simulink library "Contact_Forces_Lib"  (R2025a)
settings: Solver=ode45  StartTime=0.0  StopTime=10.0  RelTol=1e-3  EnableMultiTasking=on
undefined symbols (not defined in the file or in its folder): b_contact, custom_param_1, custom_param_2, Extr_Data_Ring, k_contact, l_cone, length_cylinder, length_tube, mu_kinetic, mu_static, pen_exponent, pen_full_damp_F, rad_s_cone, radius_cylinder, radius_tube, v_thr, X, Y, Z
libraries: nesl_utility x197, sm_lib x115, $bdroot x72, simulink x20, fl_lib x4
(part 6 of 12)

== system Contact_Forces_Lib/2D/Circle to Finite Line Force Enabled/Demux ==
  F : Inport
  Bus Creator : BusCreator  Inputs=2
  Bus Creator1 : BusCreator  Inputs=3
  Constant : Constant  Value=0
  Demux : Demux  Outputs=[3 3]
  Demux1 : Demux  Outputs=3
  Demux2 : Demux  Outputs=3
  Gain : Gain  Gain=-1
  Gain1 : Gain
  Simulink-PS Converter{,1..7} (8 alike) : nesl_utility/Simulink-PS Converter  PhysicalDomain=network_engine_domain  SubClassName=ps_input  LeftPortType=input  RightPortType=output  PseudoPeriodic=off  Frequencies=[]  NoiseDistribution=none  NoiseParameters=[]  Unit=1  AffineConversion=off  FilteringAndDerivatives=zero  SimscapeFilterOrder=1  InputFilterTimeConstant=0.005  UdotUserProvided=[]
  Fx Cir : PMIOPort  Side=Right
  Fy Cir : PMIOPort  Port=2  Side=Right
  Fz Cir : PMIOPort  Port=3  Side=Right
  Tz Cir : PMIOPort  Port=4  Side=Right
  Fx Lin : PMIOPort  Port=5  Side=Right
  Fy Lin : PMIOPort  Port=6  Side=Right
  Fz Lin : PMIOPort  Port=7  Side=Right
  Tz Lin : PMIOPort  Port=8  Side=Right
  FCir : Outport  VectorParamsAs1DForOutWhenUnconnected=off
  FLin : Outport  Port=2  VectorParamsAs1DForOutWhenUnconnected=off
  wires:
  Bus Creator1/1 -> FLin/1  "FLin"
  Bus Creator/1 -> FCir/1  "FCir"
  Gain1/1 -> Demux1/1
  F/1 -> Demux/1
  Demux/2 -> Gain/1
  Demux/1 -> Gain1/1
  Demux1/1 -> Simulink-PS Converter/1, Bus Creator/1  "Fx"
  Demux1/2 -> Simulink-PS Converter1/1, Bus Creator/2  "Fy"
  Constant/1 -> Simulink-PS Converter2/1, Simulink-PS Converter5/1
  Demux2/2 -> Simulink-PS Converter4/1, Bus Creator1/2  "Fy"
  Demux2/1 -> Simulink-PS Converter3/1, Bus Creator1/1  "Fx"
  Demux2/3 -> Simulink-PS Converter6/1, Bus Creator1/3  "Tz"
  Demux1/3 -> Simulink-PS Converter7/1
  Gain/1 -> Demux2/1
  connections:
  Fz Cir/RConn1 -- Simulink-PS Converter2/RConn1
  Fy Cir/RConn1 -- Simulink-PS Converter1/RConn1
  Fx Cir/RConn1 -- Simulink-PS Converter/RConn1
  Tz Lin/RConn1 -- Simulink-PS Converter6/RConn1
  Fx Lin/RConn1 -- Simulink-PS Converter3/RConn1
  Fy Lin/RConn1 -- Simulink-PS Converter4/RConn1
  Fz Lin/RConn1 -- Simulink-PS Converter5/RConn1
  Tz Cir/RConn1 -- Simulink-PS Converter7/RConn1

== system Contact_Forces_Lib/2D/Circle to Finite Line Force Enabled/Enable Force ==
  y : Inport
  Abs1 : Abs  ZeroCross=off  SaturateOnIntegerOverflow=off
  Activation limit for contact force : Constant  Value=line_length/2
  Sum : Sum  Inputs=+-
  Enable : Outport  VectorParamsAs1DForOutWhenUnconnected=off
  wires:
  Abs1/1 -> Sum/2
  y/1 -> Abs1/1
  Activation limit for contact force/1 -> Sum/1
  Sum/1 -> Enable/1

== system Contact_Forces_Lib/2D/Circle to Finite Line Force Enabled/Forces ==
  M arm : Inport
  X Sep : Inport  Port=2
  Pos Cmp : Inport  Port=3
  Pen : Inport  Port=4
  Vel : Inport  Port=5
  Vel_Cmp : Inport  Port=6
  Unit Vector : Inport  Port=7
  vy : Inport  Port=8
  wz : Inport  Port=9
  Action Port : ActionPort  ActionPortLabel=if { }
  Force Law : $bdroot/Force Law  SystemSampleTime=-1  LabelModeActiveChoice=Linear  VariantActivationTime=update diagram  EmptyChoice=off  PassThrough=off  PassThroughVariantControl=(default)  EmptyChoiceVariantControl=(default)  AllowFlexibleInterface=on  Latency=0  AutoFrameSizeCalculation=off
  Mux : Mux  Inputs=6
  Resolve Forces : Subsystem
  Subsystem : Subsystem
  Fnf : Outport  InitialOutput=[0]  VectorParamsAs1DForOutWhenUnconnected=off
  F : Outport  Port=2  VectorParamsAs1DForOutWhenUnconnected=off
  wires:
  Subsystem/1(Out) -> Fnf/1
  Resolve Forces/8(Ff) -> Subsystem/2(Ff)
  Resolve Forces/7(Fn) -> Subsystem/1(Fn)
  Resolve Forces/4(Fx Lin) -> Mux/4
  Pen/1 -> Force Law/1
  Vel/1 -> Force Law/2
  Resolve Forces/5(Fy Lin) -> Mux/5
  Resolve Forces/6(Tz Lin) -> Mux/6
  Resolve Forces/1(Fx Cir) -> Mux/1
  Resolve Forces/2(Fy Cir) -> Mux/2
  M arm/1 -> Resolve Forces/1(Moment arm)
  Pos Cmp/1 -> Resolve Forces/2(Pos Cmp)
  Mux/1 -> F/1
  Vel_Cmp/1 -> Resolve Forces/6(Vel Cmp)
  Unit Vector/1 -> Resolve Forces/7(Unit Vector)
  wz/1 -> Resolve Forces/9(wz)
  vy/1 -> Resolve Forces/8(vy)
  Resolve Forces/3(Tz Cir) -> Mux/3
  Force Law/1 -> Resolve Forces/4(Spr Force Mag)
  Force Law/2 -> Resolve Forces/5(Damp Force Mag)
  X Sep/1 -> Resolve Forces/3(X Sep)

== system Contact_Forces_Lib/2D/Circle to Finite Line Force Enabled/No Force ==
  Action Port : ActionPort  ActionPortLabel=else { }
  Zeros : Constant  Value=[0 0 0 0 0 0]  SampleTime=0
  Zeros1 : Constant  Value=[0 0]  SampleTime=0
  Fnf : Outport  InitialOutput=[0]  VectorParamsAs1DForOutWhenUnconnected=off
  F : Outport  Port=2  InitialOutput=[0 0 0 0 0 0]  VectorParamsAs1DForOutWhenUnconnected=off
  wires:
  Zeros1/1 -> Fnf/1
  Zeros/1 -> F/1

== system Contact_Forces_Lib/2D/Circle to Finite Line Force Enabled/Sensing ==
  In : Inport
  Bus Selector : BusSelector  OutputSignals=vy
  PS-Simulink Converter{,1..5} (6 alike) : nesl_utility/PS-Simulink Converter  PhysicalDomain=network_engine_domain  SubClassName=ps_output  LeftPortType=input  RightPortType=output  PseudoPeriodic=off  Frequencies=[]  VectorFormat=1-D array  Unit=1  AffineConversion=off
  Product : Product
  Selector : Selector  NumberOfDimensions=2  InputPortWidth=3  IndexOptions=Index vector (dialog),Index vector (dialog)  Indices=[1],[1,2]  OutputSizes=1,1
  Sign : Signum  ZeroCross=off
  Sum : Sum  Inputs=|+-
  Transform Sensor : sm_lib/Frames and Transforms/Transform Sensor  MeasurementFrame=Base  RotationSequence=XYX  SenseAngle=off  SenseAxis=off  SenseQ=off  SenseR=on  SenseRotationSequence=off  SenseOmegaX=off  SenseOmegaY=off  SenseOmegaZ=on  SenseOmega=off  SenseQDot=off  SenseRDot=off  SenseRotationSequenceDot=off  SenseAlphaX=off  SenseAlphaY=off  SenseAlphaZ=off  SenseAlpha=off  SenseQDDot=off  SenseRDDot=off  SenseX=on  SenseY=on  SenseZ=off  SenseXYZ=off  SenseRad=off  SenseAzim=off  SenseDist=off  SenseInc=off  SenseXDot=on  SenseYDot=on  SenseZDot=off  SenseXYZDot=off  SenseRadDot=off  SenseAzimDot=off  SenseDistDot=off  SenseIncDot=off  SenseXDDot=off  SenseYDDot=off  SenseZDDot=off  SenseXYZDDot=off  SenseRadDDot=off  SenseAzimDDot=off  SenseDistDDot=off  SenseIncDDot=off
  F : PMIOPort  Side=Left
  B : PMIOPort  Port=2  Side=Left
  y : Outport  VectorParamsAs1DForOutWhenUnconnected=off
  x : Outport  Port=2  VectorParamsAs1DForOutWhenUnconnected=off
  vx : Outport  Port=3  VectorParamsAs1DForOutWhenUnconnected=off
  q : Outport  Port=4  VectorParamsAs1DForOutWhenUnconnected=off
  vy : Outport  Port=5  VectorParamsAs1DForOutWhenUnconnected=off
  wz : Outport  Port=6  VectorParamsAs1DForOutWhenUnconnected=off
  wires:
  PS-Simulink Converter1/1 -> y/1
  PS-Simulink Converter2/1 -> vx/1
  PS-Simulink Converter3/1 -> Sum/1
  PS-Simulink Converter4/1 -> wz/1
  PS-Simulink Converter5/1 -> Selector/1
  Selector/1 -> q/1
  Product/1 -> Sum/2
  Sign/1 -> Product/1
  Bus Selector/1 -> Product/2  "<vy>"
  In/1 -> Bus Selector/1
  PS-Simulink Converter/1 -> x/1, Sign/1
  Sum/1 -> vy/1
  connections:
  Transform Sensor/RConn1 -- F/RConn1
  Transform Sensor/LConn1 -- B/RConn1
  PS-Simulink Converter4/LConn1 -- Transform Sensor/RConn3
  PS-Simulink Converter/LConn1 -- Transform Sensor/RConn4
  PS-Simulink Converter1/LConn1 -- Transform Sensor/RConn5
  PS-Simulink Converter2/LConn1 -- Transform Sensor/RConn6
  PS-Simulink Converter3/LConn1 -- Transform Sensor/RConn7
  PS-Simulink Converter5/LConn1 -- Transform Sensor/RConn2

== system Contact_Forces_Lib/2D/Circle to Hole Force/Calculate Penetration ==
  Pos : Inport
  Vel : Inport  Port=2
  Constant : Constant  Value=max_frame_sep
  Dead Zone Outside : DeadZone  LowerValue=-inf  UpperValue=0
  Gain2 : Gain  Gain=-1
  Sum1 : Sum  Inputs=|-+
  Pen : Outport  VectorParamsAs1DForOutWhenUnconnected=off
  Pen Vel : Outport  Port=2  VectorParamsAs1DForOutWhenUnconnected=off
  wires:
  Pos/1 -> Sum1/1
  Sum1/1 -> Dead Zone Outside/1
  Constant/1 -> Sum1/2
  Dead Zone Outside/1 -> Pen/1
  Gain2/1 -> Pen Vel/1
  Vel/1 -> Gain2/1

== system Contact_Forces_Lib/2D/Circle to Hole Force/Sensing ==
  PS-Simulink Converter1 : nesl_utility/PS-Simulink Converter  PhysicalDomain=network_engine_domain  SubClassName=ps_output  LeftPortType=input  RightPortType=output  PseudoPeriodic=off  Frequencies=[]  VectorFormat=1-D array  Unit=deg  AffineConversion=off
  PS-Simulink Converter4 : nesl_utility/PS-Simulink Converter  PhysicalDomain=network_engine_domain  SubClassName=ps_output  LeftPortType=input  RightPortType=output  PseudoPeriodic=off  Frequencies=[]  VectorFormat=1-D array  Unit=1  AffineConversion=off
  PS-Simulink Converter5 : nesl_utility/PS-Simulink Converter  PhysicalDomain=network_engine_domain  SubClassName=ps_output  LeftPortType=input  RightPortType=output  PseudoPeriodic=off  Frequencies=[]  VectorFormat=1-D array  Unit=1  AffineConversion=off
  PS-Simulink Converter6 : nesl_utility/PS-Simulink Converter  PhysicalDomain=network_engine_domain  SubClassName=ps_output  LeftPortType=input  RightPortType=output  PseudoPeriodic=off  Frequencies=[]  VectorFormat=1-D array  Unit=1  AffineConversion=off
  Selector : Selector  NumberOfDimensions=2  InputPortWidth=3  IndexOptions=Index vector (dialog),Index vector (dialog)  Indices=[1],[1,2]  OutputSizes=1,1
  Transform Sensor : sm_lib/Frames and Transforms/Transform Sensor  MeasurementFrame=NonRotatingBase  RotationSequence=XYX  SenseAngle=off  SenseAxis=off  SenseQ=off  SenseR=off  SenseRotationSequence=off  SenseOmegaX=off  SenseOmegaY=off  SenseOmegaZ=off  SenseOmega=off  SenseQDot=off  SenseRDot=off  SenseRotationSequenceDot=off  SenseAlphaX=off  SenseAlphaY=off  SenseAlphaZ=off  SenseAlpha=off  SenseQDDot=off  SenseRDDot=off  SenseX=off  SenseY=off  SenseZ=off  SenseXYZ=off  SenseRad=on  SenseAzim=on  SenseDist=off  SenseInc=off  SenseXDot=off  SenseYDot=off  SenseZDot=off  SenseXYZDot=off  SenseRadDot=on  SenseAzimDot=off  SenseDistDot=off  SenseIncDot=off  SenseXDDot=off  SenseYDDot=off  SenseZDDot=off  SenseXYZDDot=off  SenseRadDDot=off  SenseAzimDDot=off  SenseDistDDot=off  SenseIncDDot=off
  Transform Sensor1 : sm_lib/Frames and Transforms/Transform Sensor  MeasurementFrame=World  RotationSequence=XYX  SenseAngle=off  SenseAxis=off  SenseQ=off  SenseR=on  SenseRotationSequence=off  SenseOmegaX=off  SenseOmegaY=off  SenseOmegaZ=off  SenseOmega=off  SenseQDot=off  SenseRDot=off  SenseRotationSequenceDot=off  SenseAlphaX=off  SenseAlphaY=off  SenseAlphaZ=off  SenseAlpha=off  SenseQDDot=off  SenseRDDot=off  SenseX=off  SenseY=off  SenseZ=off  SenseXYZ=off  SenseRad=off  SenseAzim=off  SenseDist=off  SenseInc=off  SenseXDot=off  SenseYDot=off  SenseZDot=off  SenseXYZDot=off  SenseRadDot=off  SenseAzimDot=off  SenseDistDot=off  SenseIncDot=off  SenseXDDot=off  SenseYDDot=off  SenseZDDot=off  SenseXYZDDot=off  SenseRadDDot=off  SenseAzimDDot=off  SenseDistDDot=off  SenseIncDDot=off
  F : PMIOPort  Side=Left
  B : PMIOPort  Port=2  Side=Left
  rad : Outport  VectorParamsAs1DForOutWhenUnconnected=off
  vrad : Outport  Port=2  VectorParamsAs1DForOutWhenUnconnected=off
  q : Outport  Port=3  VectorParamsAs1DForOutWhenUnconnected=off
  azm : Outport  Port=4  VectorParamsAs1DForOutWhenUnconnected=off
  wires:
  PS-Simulink Converter1/1 -> azm/1
  PS-Simulink Converter5/1 -> rad/1
  PS-Simulink Converter4/1 -> vrad/1
  Selector/1 -> q/1
  PS-Simulink Converter6/1 -> Selector/1
  connections:
  PS-Simulink Converter4/LConn1 -- Transform Sensor/RConn4
  PS-Simulink Converter5/LConn1 -- Transform Sensor/RConn2
  PS-Simulink Converter1/LConn1 -- Transform Sensor/RConn3
  PS-Simulink Converter6/LConn1 -- Transform Sensor1/RConn2
  Transform Sensor1/LConn1 -- B/RConn1 -- Transform Sensor/LConn1
  Transform Sensor1/RConn1 -- Transform Sensor/RConn1 -- F/RConn1

== system Contact_Forces_Lib/2D/Circle to Ring Force/Check Active ==
  Force : Inport
  Active : Inport  Port=2
  PosVel : Inport  Port=3
  Bus Creator : BusCreator  Inputs=7
  Bus Selector : BusSelector  OutputSignals=Normal Force,Friction Force,Penetration,Penetration Vel,Spr Force,Damp Force
  Data Type Conversion : DataTypeConversion  OutDataTypeStr=double  SaturateOnIntegerOverflow=off  RndMeth=Floor
  Demux : Demux  Outputs=6
  Mux : Mux  Inputs=6
  Product : Product
  Out : Outport  VectorParamsAs1DForOutWhenUnconnected=off
  wires:
  Demux/1 -> Bus Creator/1  "Normal Force"
  Demux/2 -> Bus Creator/2  "Friction Force"
  Demux/3 -> Bus Creator/3  "Penetration"
  Demux/6 -> Bus Creator/6  "Damp Force"
  Demux/5 -> Bus Creator/5  "Spr Force"
  Demux/4 -> Bus Creator/4  "Penetration Vel"
  Product/1 -> Demux/1
  Data Type Conversion/1 -> Product/1
  Active/1 -> Data Type Conversion/1
  Mux/1 -> Product/2
  Bus Selector/6 -> Mux/6  "<Damp Force>"
  Bus Creator/1 -> Out/1
  Force/1 -> Bus Selector/1
  Bus Selector/5 -> Mux/5  "<Spr Force>"
  Bus Selector/3 -> Mux/3  "<Penetration>"
  Bus Selector/4 -> Mux/4  "<Penetration Vel>"
  PosVel/1 -> Bus Creator/7
  Bus Selector/2 -> Mux/2  "<Friction Force>"
  Bus Selector/1 -> Mux/1  "<Normal Force>"

== system Contact_Forces_Lib/2D/Circle to Ring Force/Check Active Range ==
  azm : Inport
  " Upper Bound" : simulink/Logic and Bit Operations/Compare To Constant  relop=<=  const=active_angle(2)  OutDataTypeStr=boolean  ZeroCross=off
  Logical Operator : Logic  AllPortsSameDT=off  OutDataTypeStr=boolean
  Lower Bound : simulink/Logic and Bit Operations/Compare To Constant  relop=>=  const=active_angle(1)  OutDataTypeStr=boolean  ZeroCross=off
  En : Outport  VectorParamsAs1DForOutWhenUnconnected=off
  wires:
  azm/1 -> " Upper Bound"/1, Lower Bound/1
  " Upper Bound"/1 -> Logical Operator/1
  Logical Operator/1 -> En/1
  Lower Bound/1 -> Logical Operator/2

== system Contact_Forces_Lib/2D/Circle to Ring Force/Forces ==
  rad : Inport
  vrad : Inport  Port=2
  azm : Inport  Port=3
  vazm : Inport  Port=4
  wzf : Inport  Port=5
  R : Inport  Port=6
  Action Port : ActionPort
  Bus Creator : BusCreator  Inputs=6
  Calculate Penetration : Subsystem
  Ff : Subsystem
  Fn : Subsystem
  Force Law : $bdroot/Force Law  SystemSampleTime=-1  LabelModeActiveChoice=Linear  VariantActivationTime=update diagram  EmptyChoice=off  PassThrough=off  PassThroughVariantControl=(default)  EmptyChoiceVariantControl=(default)  AllowFlexibleInterface=on  Latency=0  AutoFrameSizeCalculation=off
  Gain1 : Gain  Gain=-1
  Mux : Mux  Inputs=6
  Product : Product
  Sum : Subsystem
  Sum1 : Sum  Inputs=+-
  Frc : Outport  VectorParamsAs1DForOutWhenUnconnected=off
  Out : Outport  Port=2  InitialOutput=[0]  VectorParamsAs1DForOutWhenUnconnected=off
  wires:
  Bus Creator/1 -> Out/1
  Force Law/1 -> Bus Creator/4, Sum1/1  "Spr Force"
  Calculate Penetration/3(Pen Vel) -> Bus Creator/1, Force Law/2  "Penetration Vel"
  vrad/1 -> Calculate Penetration/2(vrad)
  rad/1 -> Ff/7(rad), Calculate Penetration/1(rad)
  Product/1 -> Bus Creator/5, Gain1/1  "Normal Force"
  Calculate Penetration/2(Pen) -> Bus Creator/2, Ff/6(Pen), Force Law/1  "Penetration"
  Calculate Penetration/1(sign) -> Product/1
  Force Law/2 -> Bus Creator/3, Sum1/2  "Damp Force"
  Sum1/1 -> Product/2
  Gain1/1 -> Ff/5(Fn), Fn/1(Fn)
  R/1 -> Ff/1(R), Fn/2(R)
  azm/1 -> Fn/3(azm), Ff/2(azm)
  vazm/1 -> Ff/3(vazm)
  wzf/1 -> Ff/4(wzf)
  Fn/1(FxCirF) -> Sum/1(FnxCirF)
  Fn/2(FyCirF) -> Sum/2(FnyCirF)
  Fn/3(FxCirB) -> Sum/3(FnxCirB)
  Fn/4(FyCirB) -> Sum/4(FnyCirB)
  Ff/4(FyCirB) -> Sum/8(FfyCirB)
  Ff/6(TzCirB) -> Sum/10(TzCirB)
  Ff/3(FxCirB) -> Sum/7(FfxCirB)
  Ff/5(TzCirF) -> Sum/9(TzCirF)
  Ff/1(FxCirF) -> Sum/5(FfxCirF)
  Ff/2(FyCirF) -> Sum/6(FfyCirF)
  Sum/2(FyF) -> Mux/2
  Sum/3(TzF) -> Mux/3
  Sum/1(FxF) -> Mux/1
  Sum/5(FyB) -> Mux/5
  Sum/4(FxB) -> Mux/4
  Sum/6(TzB) -> Mux/6
  Mux/1 -> Frc/1
  Ff/7(Ff) -> Bus Creator/6  "Friction Force"

== system Contact_Forces_Lib/2D/Circle to Ring Force/No Force ==
  Action Port : ActionPort
  Zeros : Constant  Value=[0 0 0 0 0 0]  SampleTime=0
  F : Outport  InitialOutput=[0]  VectorParamsAs1DForOutWhenUnconnected=off
  wires:
  Zeros/1 -> F/1

== system Contact_Forces_Lib/2D/Circle to Ring Force/Sensing ==
  PS-Simulink Converter1 : nesl_utility/PS-Simulink Converter  PhysicalDomain=network_engine_domain  SubClassName=ps_output  LeftPortType=input  RightPortType=output  PseudoPeriodic=off  Frequencies=[]  VectorFormat=1-D array  Unit=deg  AffineConversion=off
  PS-Simulink Converter{2..6} (5 alike) : nesl_utility/PS-Simulink Converter  PhysicalDomain=network_engine_domain  SubClassName=ps_output  LeftPortType=input  RightPortType=output  PseudoPeriodic=off  Frequencies=[]  VectorFormat=1-D array  Unit=1  AffineConversion=off
  Selector : Selector  NumberOfDimensions=2  InputPortWidth=3  IndexOptions=Index vector (dialog),Index vector (dialog)  Indices=[1,2],[1,2]  OutputSizes=1,1
  Transform Sensor Base : sm_lib/Frames and Transforms/Transform Sensor  MeasurementFrame=Base  RotationSequence=XYX  SenseAngle=off  SenseAxis=off  SenseQ=off  SenseR=on  SenseRotationSequence=off  SenseOmegaX=off  SenseOmegaY=off  SenseOmegaZ=on  SenseOmega=off  SenseQDot=off  SenseRDot=off  SenseRotationSequenceDot=off  SenseAlphaX=off  SenseAlphaY=off  SenseAlphaZ=off  SenseAlpha=off  SenseQDDot=off  SenseRDDot=off  SenseX=off  SenseY=off  SenseZ=off  SenseXYZ=off  SenseRad=on  SenseAzim=on  SenseDist=off  SenseInc=off  SenseXDot=off  SenseYDot=off  SenseZDot=off  SenseXYZDot=off  SenseRadDot=on  SenseAzimDot=on  SenseDistDot=off  SenseIncDot=off  SenseXDDot=off  SenseYDDot=off  SenseZDDot=off  SenseXYZDDot=off  SenseRadDDot=off  SenseAzimDDot=off  SenseDistDDot=off  SenseIncDDot=off
  F : PMIOPort  Side=Left
  B : PMIOPort  Port=2  Side=Left
  rad : Outport  VectorParamsAs1DForOutWhenUnconnected=off
  vrad : Outport  Port=2  VectorParamsAs1DForOutWhenUnconnected=off
  azm : Outport  Port=3  VectorParamsAs1DForOutWhenUnconnected=off
  vazm : Outport  Port=4  VectorParamsAs1DForOutWhenUnconnected=off
  wzf : Outport  Port=5  VectorParamsAs1DForOutWhenUnconnected=off
  R : Outport  Port=6  VectorParamsAs1DForOutWhenUnconnected=off
  wires:
  PS-Simulink Converter3/1 -> wzf/1
  PS-Simulink Converter2/1 -> vazm/1
  PS-Simulink Converter6/1 -> Selector/1
  Selector/1 -> R/1
  PS-Simulink Converter4/1 -> vrad/1
  PS-Simulink Converter5/1 -> rad/1
  PS-Simulink Converter1/1 -> azm/1
  connections:
  PS-Simulink Converter2/LConn1 -- Transform Sensor Base/RConn7
  F/RConn1 -- Transform Sensor Base/RConn1
  Transform Sensor Base/LConn1 -- B/RConn1
  PS-Simulink Converter6/LConn1 -- Transform Sensor Base/RConn2
  PS-Simulink Converter1/LConn1 -- Transform Sensor Base/RConn5
  PS-Simulink Converter5/LConn1 -- Transform Sensor Base/RConn4
  PS-Simulink Converter4/LConn1 -- Transform Sensor Base/RConn6
  PS-Simulink Converter3/LConn1 -- Transform Sensor Base/RConn3

== system Contact_Forces_Lib/2D/Circle to Ring Force/Subsystem ==
  Frc : Inport
  Demux : Demux  Outputs=6
  Simulink-PS Converter{,1..5} (6 alike) : nesl_utility/Simulink-PS Converter  PhysicalDomain=network_engine_domain  SubClassName=ps_input  LeftPortType=input  RightPortType=output  PseudoPeriodic=off  Frequencies=[]  NoiseDistribution=none  NoiseParameters=[]  Unit=1  AffineConversion=off  FilteringAndDerivatives=zero  SimscapeFilterOrder=1  InputFilterTimeConstant=0.005  UdotUserProvided=1
  FxF : PMIOPort  Side=Right
  FyF : PMIOPort  Port=2  Side=Right
  TzF : PMIOPort  Port=3  Side=Right
  FxB : PMIOPort  Port=4  Side=Right
  FyB : PMIOPort  Port=5  Side=Right
  TzB : PMIOPort  Port=6  Side=Right
  wires:
  Frc/1 -> Demux/1
  Demux/6 -> Simulink-PS Converter5/1
  Demux/5 -> Simulink-PS Converter4/1
  Demux/4 -> Simulink-PS Converter3/1
  Demux/3 -> Simulink-PS Converter2/1
  Demux/1 -> Simulink-PS Converter/1
  Demux/2 -> Simulink-PS Converter1/1
  connections:
  Simulink-PS Converter2/RConn1 -- TzF/RConn1
  Simulink-PS Converter4/RConn1 -- FyB/RConn1
  Simulink-PS Converter3/RConn1 -- FxB/RConn1
  Simulink-PS Converter5/RConn1 -- TzB/RConn1
  Simulink-PS Converter/RConn1 -- FxF/RConn1
  Simulink-PS Converter1/RConn1 -- FyF/RConn1

== system Contact_Forces_Lib/2D/Composite Forces/Box to Belt Force ==
  Spd : Inport
  Add2 : Sum
  Belt Ends : Subsystem
      mask Display:
      | image(imread('Box_to_Belt_Ends_IMAGE.jpg'));
      | port_label('LConn',1,'Bel');
      | port_label('RConn',1,'Box');
      | port_label('input',1,'In');
      | port_label('output',1,'Fn');
  Belt Faces : Subsystem
      mask Display:
      | image(imread('Box_to_Belt_Faces_IMAGE.jpg'));
      | port_label('LConn',1,'Bel');
      | port_label('RConn',1,'Box');
      | port_label('input',1,'In');
      | port_label('output',1,'Fn');
  Bus Creator : BusCreator  Inputs=2
  Enable : Constant
  Box : PMIOPort  Side=Right
  Bel : PMIOPort  Port=2  Side=Left
  Fn : Outport  VectorParamsAs1DForOutWhenUnconnected=off
  wires:
  Belt Faces/1(Fn) -> Add2/1
  Belt Ends/1(Fn) -> Add2/2
  Add2/1 -> Fn/1
  Enable/1 -> Bus Creator/1  "Enable"
  Spd/1 -> Bus Creator/2  "vy"
  Bus Creator/1 -> Belt Ends/1(In), Belt Faces/1(In1)
  connections:
  Belt Faces/LConn1 -- Bel/RConn1 -- Belt Ends/LConn1
  Belt Faces/RConn1 -- Box/RConn1 -- Belt Ends/RConn1

== system Contact_Forces_Lib/2D/Composite Forces/Box to Box Force ==
  Abs : Abs  ZeroCross=off  SaturateOnIntegerOverflow=off
  Abs1 : Abs  ZeroCross=off  SaturateOnIntegerOverflow=off
  Add : Sum
  BoxB Corners : Subsystem  mask(Contact Forces, Base Box Corners){}
      mask help:
      | This subsystem models planar contact forces the corners of the Follower box and the faces of the Base Box.
      |
      | Click the Help button for a diagram of the contact forces and the parameters.
      mask Help: web(which('Box_to_Box_Contact_Forces_BoxB_Corners.html'));
      mask Display:
      | image(imread('BoxB_Corners_IMAGE.jpg'));
      | port_label('LConn',1,'BoxB');
      | port_label('RConn',1,'BoxF');
  BoxF Corners : Subsystem  mask(Contact Forces, Follower Box Corners){}
      mask help:
      | This subsystem models planar contact forces the corners of the Follower box and the faces of the Base Box.
      |
      | Click the Help button for a diagram of the contact forces and the parameters.
      mask Help: web(which('Box_to_Box_Contact_Forces_BoxF_Corners.html'));
      mask Display:
      | image(imread('BoxF_Corners_IMAGE.jpg'));
      | port_label('LConn',1,'BoxB');
      | port_label('RConn',1,'BoxF');
  Goto Tag Visibility : GotoTagVisibility  GotoTag=FrcFC
  Goto Tag Visibility1 : GotoTagVisibility  GotoTag=FrcBC
  Sum of Elements : Sum  Inputs=+
  Sum of Elements1 : Sum  Inputs=+
  BoxF : PMIOPort  Side=Left
  BoxB : PMIOPort  Port=2  Side=Right
  Out : Outport  VectorParamsAs1DForOutWhenUnconnected=off
  wires:
  Sum of Elements1/1 -> Add/2
  Add/1 -> Out/1
  Abs1/1 -> Sum of Elements1/1
  [FrcBC] -> Abs1/1
  Abs/1 -> Sum of Elements/1
  Sum of Elements/1 -> Add/1
  [FrcFC] -> Abs/1
  connections:
  BoxB Corners/LConn1 -- BoxF Corners/LConn1 -- BoxB/RConn1
  BoxB Corners/RConn1 -- BoxF Corners/RConn1 -- BoxF/RConn1

== system Contact_Forces_Lib/3D/Composite Forces/Face to Belt Faces Force ==
  In : Inport
  Bus Creator : BusCreator  Inputs=4
  Sphere to Plane Force Enabled nz{1..4} (4 alike) : $bdroot/3D/Sphere to Plane Force Enabled  sphere_rad=FacF_rSph  plane_lenx=PlaB_x  plane_leny=PlaB_y  plane_depth=PlaB_z  force_law=Linear  k_contact=k_contact_pla2pla  b_contact=b_contact_pla2pla  pen_full_damp_F=pen_full_damp_F_pla2pla  pen_exponent=pen_exponent_pla2pla  custom_param_1=1  custom_param_2=1  friction_law=Stick-Slip Continuous  mu_kinetic=mu_kinetic_pla2pla  mu_static=mu_static_pla2pla  v_thr=v_thr_pla2pla  vis_on=off  vis_opc_en=0  vis_len_plaBz=vis_len_plaLz  vis_clr=vis_clr  vis_opc=vis_opc
  Transform Fnz1 : sm_lib/Frames and Transforms/Rigid Transform  RotationMethod=None  FollAlignAxisA=+X  BaseAlignAxisA=+Y  FollAlignAxisB=+Y  BaseAlignAxisB=+Z  RotationStandardAxis=+Z  RotationAngle=0.0  RotationAngleUnits=deg  RotationArbitraryAxis=[0 0 1]  RotationSequenceAxes=FollowerAxes  RotationSequence=XYX  RotationSequenceAngles=[0 0 0]  RotationSequenceAnglesUnits=deg  RotationMatrix=[1 0 0; 0 1 0; 0 0 1]  Quaternion=[1 0 0 0]  TranslationMethod=Cartesian  TranslationCartesianOffset=[FacF_x/2 FacF_y/2 -FacF_z]+[-1 -1 1*sign(FacF_z)]*FacF_rSph  TranslationCartesianOffsetUnits=m  TranslationStandardAxis=-Z  TranslationStandardOffset=0  TranslationStandardOffsetUnits=m  TranslationROffset=0  TranslationROffsetUnits=m  TranslationThetaOffset=0  TranslationThetaOffsetUnits=deg  TranslationZOffset=0  TranslationZOffsetUnits=m
  Transform Fnz2 : sm_lib/Frames and Transforms/Rigid Transform  RotationMethod=None  FollAlignAxisA=+X  BaseAlignAxisA=+Y  FollAlignAxisB=+Y  BaseAlignAxisB=+Z  RotationStandardAxis=+Z  RotationAngle=0.0  RotationAngleUnits=deg  RotationArbitraryAxis=[0 0 1]  RotationSequenceAxes=FollowerAxes  RotationSequence=XYX  RotationSequenceAngles=[0 0 0]  RotationSequenceAnglesUnits=deg  RotationMatrix=[1 0 0; 0 1 0; 0 0 1]  Quaternion=[1 0 0 0]  TranslationMethod=Cartesian  TranslationCartesianOffset=[FacF_x/2 -FacF_y/2 -FacF_z]+[-1 1 1*sign(FacF_z)]*FacF_rSph  TranslationCartesianOffsetUnits=m  TranslationStandardAxis=-Z  TranslationStandardOffset=0  TranslationStandardOffsetUnits=m  TranslationROffset=0  TranslationROffsetUnits=m  TranslationThetaOffset=0  TranslationThetaOffsetUnits=deg  TranslationZOffset=0  TranslationZOffsetUnits=m
  Transform Fnz3 : sm_lib/Frames and Transforms/Rigid Transform  RotationMethod=None  FollAlignAxisA=+X  BaseAlignAxisA=+Y  FollAlignAxisB=+Y  BaseAlignAxisB=+Z  RotationStandardAxis=+Z  RotationAngle=0.0  RotationAngleUnits=deg  RotationArbitraryAxis=[0 0 1]  RotationSequenceAxes=FollowerAxes  RotationSequence=XYX  RotationSequenceAngles=[0 0 0]  RotationSequenceAnglesUnits=deg  RotationMatrix=[1 0 0; 0 1 0; 0 0 1]  Quaternion=[1 0 0 0]  TranslationMethod=Cartesian  TranslationCartesianOffset=[-FacF_x/2 -FacF_y/2 -FacF_z]+[1 1 1*sign(FacF_z)]*FacF_rSph  TranslationCartesianOffsetUnits=m  TranslationStandardAxis=-Z  TranslationStandardOffset=0  TranslationStandardOffsetUnits=m  TranslationROffset=0  TranslationROffsetUnits=m  TranslationThetaOffset=0  TranslationThetaOffsetUnits=deg  TranslationZOffset=0  TranslationZOffsetUnits=m
  Transform Fnz4 : sm_lib/Frames and Transforms/Rigid Transform  RotationMethod=None  FollAlignAxisA=+X  BaseAlignAxisA=+Y  FollAlignAxisB=+Y  BaseAlignAxisB=+Z  RotationStandardAxis=+Z  RotationAngle=0.0  RotationAngleUnits=deg  RotationArbitraryAxis=[0 0 1]  RotationSequenceAxes=FollowerAxes  RotationSequence=XYX  RotationSequenceAngles=[0 0 0]  RotationSequenceAnglesUnits=deg  RotationMatrix=[1 0 0; 0 1 0; 0 0 1]  Quaternion=[1 0 0 0]  TranslationMethod=Cartesian  TranslationCartesianOffset=[-FacF_x/2 FacF_y/2 -FacF_z]+[1 -1 1*sign(FacF_z)]*FacF_rSph  TranslationCartesianOffsetUnits=m  TranslationStandardAxis=-Z  TranslationStandardOffset=0  TranslationStandardOffsetUnits=m  TranslationROffset=0  TranslationROffsetUnits=m  TranslationThetaOffset=0  TranslationThetaOffsetUnits=deg  TranslationZOffset=0  TranslationZOffsetUnits=m
  PlaB : PMIOPort  Side=Right
  FacF : PMIOPort  Port=2  Side=Left
  Out : Outport  VectorParamsAs1DForOutWhenUnconnected=off
  wires:
  In/1 -> Sphere to Plane Force Enabled nz4/1, Sphere to Plane Force Enabled nz3/1, Sphere to Plane Force Enabled nz2/1, Sphere to Plane Force Enabled nz1/1
  Bus Creator/1 -> Out/1
  Sphere to Plane Force Enabled nz3/1 -> Bus Creator/3  "fz3"
  Sphere to Plane Force Enabled nz1/1 -> Bus Creator/1  "fz1"
  Sphere to Plane Force Enabled nz2/1 -> Bus Creator/2  "fz2"
  Sphere to Plane Force Enabled nz4/1 -> Bus Creator/4  "fz4"
  connections:
  Sphere to Plane Force Enabled nz3/LConn1 -- Transform Fnz3/RConn1
  Sphere to Plane Force Enabled nz2/LConn1 -- Transform Fnz2/RConn1
  Sphere to Plane Force Enabled nz4/LConn1 -- Transform Fnz4/RConn1
  Sphere to Plane Force Enabled nz1/LConn1 -- Transform Fnz1/RConn1
  Sphere to Plane Force Enabled nz4/RConn1 -- Sphere to Plane Force Enabled nz2/RConn1 -- Sphere to Plane Force Enabled nz1/RConn1 -- PlaB/RConn1 -- Sphere to Plane Force Enabled nz3/RConn1
  Transform Fnz1/LConn1 -- Transform Fnz3/LConn1 -- Transform Fnz4/LConn1 -- FacF/RConn1 -- Transform Fnz2/LConn1

== system Contact_Forces_Lib/3D/Composite Forces/Face to Plane Force ==
  Bus Creator : BusCreator  Inputs=4
  Sphere to Plane Force nz{1..4} (4 alike) : $bdroot/3D/Sphere to Plane Force  sphere_rad=FacF_rSph  plane_lenx=PlaB_x  plane_leny=PlaB_y  plane_depth=PlaB_z  force_law=Linear  k_contact=k_contact_pla2pla  b_contact=b_contact_pla2pla  pen_full_damp_F=pen_full_damp_F_pla2pla  pen_exponent=pen_exponent_pla2pla  custom_param_1=1  custom_param_2=1  friction_law=None  mu_kinetic=mu_kinetic_pla2pla  mu_static=mu_static_pla2pla  v_thr=v_thr_pla2pla  vis_on=off  vis_opc_en=0  vis_len_plaBz=vis_len_plaLz  vis_clr=vis_clr  vis_opc=vis_opc
  Transform Fnz1 : sm_lib/Frames and Transforms/Rigid Transform  RotationMethod=None  FollAlignAxisA=+X  BaseAlignAxisA=+Y  FollAlignAxisB=+Y  BaseAlignAxisB=+Z  RotationStandardAxis=+Z  RotationAngle=0.0  RotationAngleUnits=deg  RotationArbitraryAxis=[0 0 1]  RotationSequenceAxes=FollowerAxes  RotationSequence=XYX  RotationSequenceAngles=[0 0 0]  RotationSequenceAnglesUnits=deg  RotationMatrix=[1 0 0; 0 1 0; 0 0 1]  Quaternion=[1 0 0 0]  TranslationMethod=Cartesian  TranslationCartesianOffset=[FacF_x/2 FacF_y/2 -FacF_z]+[-1 -1 1*sign(FacF_z)]*FacF_rSph  TranslationCartesianOffsetUnits=m  TranslationStandardAxis=-Z  TranslationStandardOffset=0  TranslationStandardOffsetUnits=m  TranslationROffset=0  TranslationROffsetUnits=m  TranslationThetaOffset=0  TranslationThetaOffsetUnits=deg  TranslationZOffset=0  TranslationZOffsetUnits=m
  Transform Fnz2 : sm_lib/Frames and Transforms/Rigid Transform  RotationMethod=None  FollAlignAxisA=+X  BaseAlignAxisA=+Y  FollAlignAxisB=+Y  BaseAlignAxisB=+Z  RotationStandardAxis=+Z  RotationAngle=0.0  RotationAngleUnits=deg  RotationArbitraryAxis=[0 0 1]  RotationSequenceAxes=FollowerAxes  RotationSequence=XYX  RotationSequenceAngles=[0 0 0]  RotationSequenceAnglesUnits=deg  RotationMatrix=[1 0 0; 0 1 0; 0 0 1]  Quaternion=[1 0 0 0]  TranslationMethod=Cartesian  TranslationCartesianOffset=[FacF_x/2 -FacF_y/2 -FacF_z]+[-1 1 1*sign(FacF_z)]*FacF_rSph  TranslationCartesianOffsetUnits=m  TranslationStandardAxis=-Z  TranslationStandardOffset=0  TranslationStandardOffsetUnits=m  TranslationROffset=0  TranslationROffsetUnits=m  TranslationThetaOffset=0  TranslationThetaOffsetUnits=deg  TranslationZOffset=0  TranslationZOffsetUnits=m
  Transform Fnz3 : sm_lib/Frames and Transforms/Rigid Transform  RotationMethod=None  FollAlignAxisA=+X  BaseAlignAxisA=+Y  FollAlignAxisB=+Y  BaseAlignAxisB=+Z  RotationStandardAxis=+Z  RotationAngle=0.0  RotationAngleUnits=deg  RotationArbitraryAxis=[0 0 1]  RotationSequenceAxes=FollowerAxes  RotationSequence=XYX  RotationSequenceAngles=[0 0 0]  RotationSequenceAnglesUnits=deg  RotationMatrix=[1 0 0; 0 1 0; 0 0 1]  Quaternion=[1 0 0 0]  TranslationMethod=Cartesian  TranslationCartesianOffset=[-FacF_x/2 -FacF_y/2 -FacF_z]+[1 1 1*sign(FacF_z)]*FacF_rSph  TranslationCartesianOffsetUnits=m  TranslationStandardAxis=-Z  TranslationStandardOffset=0  TranslationStandardOffsetUnits=m  TranslationROffset=0  TranslationROffsetUnits=m  TranslationThetaOffset=0  TranslationThetaOffsetUnits=deg  TranslationZOffset=0  TranslationZOffsetUnits=m
  Transform Fnz4 : sm_lib/Frames and Transforms/Rigid Transform  RotationMethod=None  FollAlignAxisA=+X  BaseAlignAxisA=+Y  FollAlignAxisB=+Y  BaseAlignAxisB=+Z  RotationStandardAxis=+Z  RotationAngle=0.0  RotationAngleUnits=deg  RotationArbitraryAxis=[0 0 1]  RotationSequenceAxes=FollowerAxes  RotationSequence=XYX  RotationSequenceAngles=[0 0 0]  RotationSequenceAnglesUnits=deg  RotationMatrix=[1 0 0; 0 1 0; 0 0 1]  Quaternion=[1 0 0 0]  TranslationMethod=Cartesian  TranslationCartesianOffset=[-FacF_x/2 FacF_y/2 -FacF_z]+[1 -1 1*sign(FacF_z)]*FacF_rSph  TranslationCartesianOffsetUnits=m  TranslationStandardAxis=-Z  TranslationStandardOffset=0  TranslationStandardOffsetUnits=m  TranslationROffset=0  TranslationROffsetUnits=m  TranslationThetaOffset=0  TranslationThetaOffsetUnits=deg  TranslationZOffset=0  TranslationZOffsetUnits=m
  PlaB : PMIOPort  Side=Right
  FacF : PMIOPort  Port=2  Side=Left
  Out : Outport  VectorParamsAs1DForOutWhenUnconnected=off
  wires:
  Sphere to Plane Force nz4/1 -> Bus Creator/4  "fz4"
  Sphere to Plane Force nz2/1 -> Bus Creator/2  "fz2"
  Sphere to Plane Force nz1/1 -> Bus Creator/1  "fz1"
  Sphere to Plane Force nz3/1 -> Bus Creator/3  "fz3"
  Bus Creator/1 -> Out/1
  connections:
  FacF/RConn1 -- Transform Fnz1/LConn1 -- Transform Fnz2/LConn1 -- Transform Fnz4/LConn1 -- Transform Fnz3/LConn1
  Sphere to Plane Force nz4/RConn1 -- Sphere to Plane Force nz3/RConn1 -- PlaB/RConn1 -- Sphere to Plane Force nz2/RConn1 -- Sphere to Plane Force nz1/RConn1
  Sphere to Plane Force nz1/LConn1 -- Transform Fnz1/RConn1
  Sphere to Plane Force nz4/LConn1 -- Transform Fnz4/RConn1
  Sphere to Plane Force nz2/LConn1 -- Transform Fnz2/RConn1
  Sphere to Plane Force nz3/LConn1 -- Transform Fnz3/RConn1

== system Contact_Forces_Lib/3D/Composite Forces/Sphere to Belt Force ==
  In : Inport
  Bus Creator : BusCreator  Inputs=3
  Force BeltF to Sph : $bdroot/3D/Sphere to Tube Force Enabled  radius_sphere=sph_rad  radius_tube=belt_h/2*0.8  d_tube=belt_h*0.2  l_tube=belt_w  active_angle=[-90 90]  force_law=Linear  k_contact=k_contact_sph2bel  b_contact=b_contact_sph2bel  pen_full_damp_F=pen_full_damp_F_sph2bel  pen_exponent=pen_exponent_sph2bel  custom_param_1=1  custom_param_2=1  friction_law=Stick-Slip Continuous  mu_kinetic=mu_kinetic_sph2bel  mu_static=mu_static_sph2bel  v_thr=v_thr_sph2bel  vis_on=off  vis_opc_en=0  vis_len_tubBx=vis_depth_sph2bel  vis_clr=vis_clr  vis_opc=vis_opc
  Force BeltM to Sph : $bdroot/3D/Sphere to Plane Force Enabled  sphere_rad=sph_rad  plane_lenx=belt_l  plane_leny=belt_w  plane_depth=belt_h/2  force_law=Linear  k_contact=k_contact_sph2bel  b_contact=b_contact_sph2bel  pen_full_damp_F=pen_full_damp_F_sph2bel  pen_exponent=pen_exponent_sph2bel  custom_param_1=1  custom_param_2=1  friction_law=Stick-Slip Continuous  mu_kinetic=mu_kinetic_sph2bel  mu_static=mu_static_sph2bel  v_thr=v_thr_sph2bel  vis_on=off  vis_opc_en=0  vis_len_plaBz=vis_depth_sph2bel  vis_clr=vis_clr  vis_opc=vis_opc
  Force BeltR to Sph : $bdroot/3D/Sphere to Tube Force Enabled  radius_sphere=sph_rad  radius_tube=belt_h/2*0.8  d_tube=belt_h*0.2  l_tube=belt_w  active_angle=[-90 90]  force_law=Linear  k_contact=k_contact_sph2bel  b_contact=b_contact_sph2bel  pen_full_damp_F=pen_full_damp_F_sph2bel  pen_exponent=pen_exponent_sph2bel  custom_param_1=1  custom_param_2=1  friction_law=Stick-Slip Continuous  mu_kinetic=mu_kinetic_sph2bel  mu_static=mu_static_sph2bel  v_thr=v_thr_sph2bel  vis_on=off  vis_opc_en=0  vis_len_tubBx=vis_depth_sph2bel  vis_clr=vis_clr  vis_opc=vis_opc
  Transform Front : sm_lib/Frames and Transforms/Rigid Transform  RotationMethod=StandardAxis  FollAlignAxisA=+X  BaseAlignAxisA=+Y  FollAlignAxisB=+Y  BaseAlignAxisB=+Z  RotationStandardAxis=+X  RotationAngle=-90  RotationAngleUnits=deg  RotationArbitraryAxis=[0 0 1]  RotationSequenceAxes=FollowerAxes  RotationSequence=XYX  RotationSequenceAngles=[0 0 0]  RotationSequenceAnglesUnits=deg  RotationMatrix=[1 0 0; 0 1 0; 0 0 1]  Quaternion=[1 0 0 0]  TranslationMethod=StandardAxis  TranslationCartesianOffset=[0 0 0]  TranslationCartesianOffsetUnits=m  TranslationStandardAxis=+X  TranslationStandardOffset=belt_l/2  TranslationStandardOffsetUnits=m  TranslationROffset=0  TranslationROffsetUnits=m  TranslationThetaOffset=0  TranslationThetaOffsetUnits=deg  TranslationZOffset=0  TranslationZOffsetUnits=m
  Transform Rear : sm_lib/Frames and Transforms/Rigid Transform  RotationMethod=RotationSequence  FollAlignAxisA=+X  BaseAlignAxisA=+Y  FollAlignAxisB=+Y  BaseAlignAxisB=+Z  RotationStandardAxis=+Y  RotationAngle=180  RotationAngleUnits=deg  RotationArbitraryAxis=[0 0 1]  RotationSequenceAxes=FollowerAxes  RotationSequence=XZX  RotationSequenceAngles=[-90 180 0]  RotationSequenceAnglesUnits=deg  RotationMatrix=[1 0 0; 0 1 0; 0 0 1]  Quaternion=[1 0 0 0]  TranslationMethod=StandardAxis  TranslationCartesianOffset=[0 0 0]  TranslationCartesianOffsetUnits=m  TranslationStandardAxis=+X  TranslationStandardOffset=-belt_l/2  TranslationStandardOffsetUnits=m  TranslationROffset=0  TranslationROffsetUnits=m  TranslationThetaOffset=0  TranslationThetaOffsetUnits=deg  TranslationZOffset=0  TranslationZOffsetUnits=m
  SphF : PMIOPort  Side=Left
  BelB : PMIOPort  Port=2  Side=Right
  Out : Outport  VectorParamsAs1DForOutWhenUnconnected=off
  wires:
  Bus Creator/1 -> Out/1
  Force BeltR to Sph/1 -> Bus Creator/3  "fRea"
  Force BeltM to Sph/1 -> Bus Creator/2  "fMid"
  In/1 -> Force BeltF to Sph/1, Force BeltM to Sph/1, Force BeltR to Sph/1
  Force BeltF to Sph/1 -> Bus Creator/1  "fFro"
  connections:
  Force BeltR to Sph/RConn1 -- Transform Rear/RConn1
  Transform Rear/LConn1 -- Force BeltM to Sph/RConn1 -- Transform Front/LConn1 -- BelB/RConn1
  Transform Front/RConn1 -- Force BeltF to Sph/RConn1
  Force BeltR to Sph/LConn1 -- Force BeltF to Sph/LConn1 -- Force BeltM to Sph/LConn1 -- SphF/RConn1

== system Contact_Forces_Lib/3D/Prototype/Cone in Ring Force ==
  Enable : Subsystem
  External Force and Torque : sm_lib/Forces and Torques/External Force and Torque  EnableForceX=off  EnableForceY=off  EnableForceZ=off  EnableForce=on  ForceResolutionFrame=AttachedFrame  EnableTorqueX=off  EnableTorqueY=off  EnableTorqueZ=off  EnableTorque=on  TorqueResolutionFrame=AttachedFrame
  If : If  IfExpression=u1
  If Action Subsystem : Subsystem  TreatAsAtomicUnit=on
  Merge : Merge
  Merge1 : Merge
  PS-Simulink Converter{1..3,5} (4 alike) : nesl_utility/PS-Simulink Converter  PhysicalDomain=network_engine_domain  SubClassName=ps_output  LeftPortType=input  RightPortType=output  PseudoPeriodic=off  Frequencies=[]  VectorFormat=1-D array  Unit=1  AffineConversion=off
  Point of Contact calc : Subsystem
  Simulink-PS Converter : nesl_utility/Simulink-PS Converter  PhysicalDomain=network_engine_domain  SubClassName=ps_input  LeftPortType=input  RightPortType=output  PseudoPeriodic=off  Frequencies=[]  NoiseDistribution=none  NoiseParameters=[]  Unit=1  AffineConversion=off  FilteringAndDerivatives=zero  SimscapeFilterOrder=1  InputFilterTimeConstant=0.005  UdotUserProvided=1
  Simulink-PS Converter1 : nesl_utility/Simulink-PS Converter  PhysicalDomain=network_engine_domain  SubClassName=ps_input  LeftPortType=input  RightPortType=output  PseudoPeriodic=off  Frequencies=[]  NoiseDistribution=none  NoiseParameters=[]  Unit=1  AffineConversion=off  FilteringAndDerivatives=zero  SimscapeFilterOrder=1  InputFilterTimeConstant=0.005  UdotUserProvided=1
  Transform Sensor : sm_lib/Frames and Transforms/Transform Sensor  MeasurementFrame=Base  RotationSequence=XYX  SenseAngle=off  SenseAxis=off  SenseQ=off  SenseR=on  SenseRotationSequence=off  SenseOmegaX=off  SenseOmegaY=off  SenseOmegaZ=off  SenseOmega=off  SenseQDot=off  SenseRDot=off  SenseRotationSequenceDot=off  SenseAlphaX=off  SenseAlphaY=off  SenseAlphaZ=off  SenseAlpha=off  SenseQDDot=off  SenseRDDot=off  SenseX=on  SenseY=on  SenseZ=on  SenseXYZ=off  SenseRad=off  SenseAzim=off  SenseDist=off  SenseInc=off  SenseXDot=off  SenseYDot=off  SenseZDot=off  SenseXYZDot=off  SenseRadDot=off  SenseAzimDot=off  SenseDistDot=off  SenseIncDot=off  SenseXDDot=off  SenseYDDot=off  SenseZDDot=off  SenseXYZDDot=off  SenseRadDDot=off  SenseAzimDDot=off  SenseDistDDot=off  SenseIncDDot=off
  B : PMIOPort  Side=Left
  F : PMIOPort  Port=2  Side=Right
  wires:
  PS-Simulink Converter2/1 -> Point of Contact calc/2(x)
  PS-Simulink Converter3/1 -> Point of Contact calc/3(y)
  PS-Simulink Converter5/1 -> Point of Contact calc/4(z), Enable/1(z)
  PS-Simulink Converter1/1 -> Point of Contact calc/1(R), Enable/2(R)
  Enable/1(Enable) -> If/1
  If/1 -> Point of Contact calc/Action
  If/2 -> If Action Subsystem/Action
  If Action Subsystem/1(F) -> Merge/1
  If Action Subsystem/2(T) -> Merge1/1
  Point of Contact calc/1(F) -> Merge/2
  Point of Contact calc/2(T) -> Merge1/2
  Merge/1 -> Simulink-PS Converter/1
  Merge1/1 -> Simulink-PS Converter1/1
  connections:
  Transform Sensor/LConn1 -- B/RConn1
  PS-Simulink Converter1/LConn1 -- Transform Sensor/RConn2
  PS-Simulink Converter2/LConn1 -- Transform Sensor/RConn3
  PS-Simulink Converter3/LConn1 -- Transform Sensor/RConn4
  PS-Simulink Converter5/LConn1 -- Transform Sensor/RConn5
  External Force and Torque/LConn1 -- Simulink-PS Converter/RConn1
  Simulink-PS Converter1/RConn1 -- External Force and Torque/LConn2
  External Force and Torque/RConn1 -- Transform Sensor/RConn1 -- F/RConn1

== system Contact_Forces_Lib/3D/Prototype/Cylinder In Ring Force ==
  Bus Creator : BusCreator  Inputs=1
  Enable : Subsystem
  External Force and Torque : sm_lib/Forces and Torques/External Force and Torque  EnableForceX=off  EnableForceY=off  EnableForceZ=off  EnableForce=on  ForceResolutionFrame=AttachedFrame  EnableTorqueX=off  EnableTorqueY=off  EnableTorqueZ=off  EnableTorque=on  TorqueResolutionFrame=AttachedFrame
  If : If  IfExpression=u1
  If Action Subsystem : Subsystem  TreatAsAtomicUnit=on
  Merge : Merge
  Merge1 : Merge
  PS-Simulink Converter{1..5} (5 alike) : nesl_utility/PS-Simulink Converter  PhysicalDomain=network_engine_domain  SubClassName=ps_output  LeftPortType=input  RightPortType=output  PseudoPeriodic=off  Frequencies=[]  VectorFormat=1-D array  Unit=1  AffineConversion=off
  Point of Contact calc : Subsystem
  Simulink-PS Converter : nesl_utility/Simulink-PS Converter  PhysicalDomain=network_engine_domain  SubClassName=ps_input  LeftPortType=input  RightPortType=output  PseudoPeriodic=off  Frequencies=[]  NoiseDistribution=none  NoiseParameters=[]  Unit=1  AffineConversion=off  FilteringAndDerivatives=zero  SimscapeFilterOrder=1  InputFilterTimeConstant=0.005  UdotUserProvided=1
  Simulink-PS Converter1 : nesl_utility/Simulink-PS Converter  PhysicalDomain=network_engine_domain  SubClassName=ps_input  LeftPortType=input  RightPortType=output  PseudoPeriodic=off  Frequencies=[]  NoiseDistribution=none  NoiseParameters=[]  Unit=1  AffineConversion=off  FilteringAndDerivatives=zero  SimscapeFilterOrder=1  InputFilterTimeConstant=0.005  UdotUserProvided=1
  Transform Sensor : sm_lib/Frames and Transforms/Transform Sensor  MeasurementFrame=Base  RotationSequence=XYX  SenseAngle=off  SenseAxis=off  SenseQ=off  SenseR=on  SenseRotationSequence=off  SenseOmegaX=off  SenseOmegaY=off  SenseOmegaZ=off  SenseOmega=off  SenseQDot=off  SenseRDot=off  SenseRotationSequenceDot=off  SenseAlphaX=off  SenseAlphaY=off  SenseAlphaZ=off  SenseAlpha=off  SenseQDDot=off  SenseRDDot=off  SenseX=on  SenseY=on  SenseZ=on  SenseXYZ=off  SenseRad=off  SenseAzim=off  SenseDist=off  SenseInc=off  SenseXDot=off  SenseYDot=off  SenseZDot=on  SenseXYZDot=off  SenseRadDot=off  SenseAzimDot=off  SenseDistDot=off  SenseIncDot=off  SenseXDDot=off  SenseYDDot=off  SenseZDDot=off  SenseXYZDDot=off  SenseRadDDot=off  SenseAzimDDot=off  SenseDistDDot=off  SenseIncDDot=off
  B : PMIOPort  Side=Left
  F : PMIOPort  Port=2  Side=Right
  Out : Outport  VectorParamsAs1DForOutWhenUnconnected=off
  wires:
  PS-Simulink Converter2/1 -> Point of Contact calc/2(x)
  PS-Simulink Converter3/1 -> Point of Contact calc/3(y)
  PS-Simulink Converter5/1 -> Point of Contact calc/4(z), Enable/1(z)
  PS-Simulink Converter1/1 -> Enable/2(R), Point of Contact calc/1(R)
  Enable/1(Enable) -> If/1
  If/1 -> Point of Contact calc/Action
  If/2 -> If Action Subsystem/Action
  If Action Subsystem/1(F) -> Merge/1
  If Action Subsystem/2(T) -> Merge1/1
  Point of Contact calc/1(F) -> Merge/2
  Point of Contact calc/2(T) -> Merge1/2
  Merge/1 -> Simulink-PS Converter/1
  Merge1/1 -> Simulink-PS Converter1/1
  PS-Simulink Converter4/1 -> Point of Contact calc/5(vz)
  Bus Creator/1 -> Out/1
  Point of Contact calc/3(pen) -> Bus Creator/1  "Penetration"
  connections:
  Transform Sensor/LConn1 -- B/RConn1
  PS-Simulink Converter1/LConn1 -- Transform Sensor/RConn2
  PS-Simulink Converter2/LConn1 -- Transform Sensor/RConn3
  PS-Simulink Converter3/LConn1 -- Transform Sensor/RConn4
  PS-Simulink Converter5/LConn1 -- Transform Sensor/RConn5
  External Force and Torque/LConn1 -- Simulink-PS Converter/RConn1
  Simulink-PS Converter1/RConn1 -- External Force and Torque/LConn2
  External Force and Torque/RConn1 -- F/RConn1 -- Transform Sensor/RConn1
  PS-Simulink Converter4/LConn1 -- Transform Sensor/RConn6

== system Contact_Forces_Lib/3D/Sphere in Sphere Force/Calculate Penetration ==
  dst : Inport
  vdst : Inport  Port=2
  Constant : Constant  Value=sphB_rad-sphF_rad
  Dead Zone : DeadZone  LowerValue=-inf  UpperValue=0
  Gain : Gain
  Sum : Sum  Inputs=-+
  Pen : Outport  VectorParamsAs1DForOutWhenUnconnected=off
  Pen Vel : Outport  Port=2  VectorParamsAs1DForOutWhenUnconnected=off
  wires:
  vdst/1 -> Gain/1
  Dead Zone/1 -> Pen/1
  dst/1 -> Sum/2
  Sum/1 -> Dead Zone/1
  Constant/1 -> Sum/1
  Gain/1 -> Pen Vel/1

== system Contact_Forces_Lib/3D/Sphere in Sphere Force/Ff ==
  Fn : Inport
  R : Inport  Port=2
  dvect : Inport  Port=3
  v : Inport  Port=4
  w : Inport  Port=5
  Check w or v non zero : Subsystem
  Cross Product : $bdroot/Math/Cross Product  SystemSampleTime=-1  VariantActivationTime=update diagram  EmptyChoice=off  PassThrough=off  PassThroughVariantControl=(default)  EmptyChoiceVariantControl=(default)  AllowFlexibleInterface=on  Latency=0  AutoFrameSizeCalculation=off
  Cross Product1 : $bdroot/Math/Cross Product  SystemSampleTime=-1  VariantActivationTime=update diagram  EmptyChoice=off  PassThrough=off  PassThroughVariantControl=(default)  EmptyChoiceVariantControl=(default)  AllowFlexibleInterface=on  Latency=0  AutoFrameSizeCalculation=off
  Friction Law : $bdroot/Friction Law  SystemSampleTime=-1  LabelModeActiveChoice=Stick_Slip_C  VariantActivationTime=update diagram  EmptyChoice=off  PassThrough=off  PassThroughVariantControl=(default)  EmptyChoiceVariantControl=(default)  AllowFlexibleInterface=on  Latency=0  AutoFrameSizeCalculation=off
  Fx1 : Constant  Value=sphB_rad
  Fx2 : Constant  Value=sphF_rad
  Gain1 : Gain  Gain=-1
  Gain2 : Gain
  Gain3 : Gain
  Merge : Merge
  Merge1 : Merge
  Product : Product
  Product1 : Product
  Product2 : Product  Inputs=/*  Multiplication=Matrix(*)
  Product3 : Product
  Product4 : Product  Inputs=/*  Multiplication=Matrix(*)
  SlipVel : Subsystem
  mag : Subsystem
  FSphF : Outport  VectorParamsAs1DForOutWhenUnconnected=off
  TSphF : Outport  Port=2  VectorParamsAs1DForOutWhenUnconnected=off
  FSphB : Outport  Port=3  VectorParamsAs1DForOutWhenUnconnected=off
  TSphB : Outport  Port=4  VectorParamsAs1DForOutWhenUnconnected=off
  Ff : Outport  Port=5  VectorParamsAs1DForOutWhenUnconnected=off
  wires:
  Check w or v non zero/2(else uv is 0) -> Merge1/2
  Check w or v non zero/1(else v is 0) -> Merge/1
  Check w or v non zero/3(Use SlipVel) -> SlipVel/Action
  Product4/1 -> FSphF/1
  R/1 -> Product4/1, Product2/1
  Cross Product1/1 -> Product2/2
  dvect/1 -> Gain2/1, Gain3/1, SlipVel/3(dvect)
  Gain1/1 -> Product4/2, Cross Product1/2
  Fx2/1 -> Product/2
  Gain3/1 -> Product/1
  Product/1 -> Cross Product1/1
  Product2/1 -> TSphF/1
  Product3/1 -> FSphB/1, Gain1/1, Cross Product/2
  Cross Product/1 -> TSphB/1
  Product1/1 -> Cross Product/1
  Fx1/1 -> Product1/2
  Gain2/1 -> Product1/1
  v/1 -> Check w or v non zero/2(v), SlipVel/2(v)
  w/1 -> Check w or v non zero/1(w), SlipVel/1(w)
  Friction Law/1 -> Product3/1, Ff/1
  mag/1(mag) -> Friction Law/1
  Fn/1 -> mag/1(vect)
  SlipVel/1(vabs) -> Merge/2
  SlipVel/2(vuvect) -> Merge1/1
  Merge/1 -> Friction Law/2
  Merge1/1 -> Product3/2

== system Contact_Forces_Lib/3D/Sphere in Sphere Force/Fn ==
  R : Inport
  SprF : Inport  Port=2
  DamF : Inport  Port=3
  dvect : Inport  Port=4
  Gain : Gain  Gain=-1
  Gain1 : Gain  Gain=-1
  Product : Product
  Product2 : Product  Inputs=/*  Multiplication=Matrix(*)
  Sum : Sum  Inputs=|+-
  Fn : Outport  VectorParamsAs1DForOutWhenUnconnected=off
  FSphF : Outport  Port=2  VectorParamsAs1DForOutWhenUnconnected=off
  FSphB : Outport  Port=3  VectorParamsAs1DForOutWhenUnconnected=off
  wires:
  SprF/1 -> Sum/1
  DamF/1 -> Sum/2
  R/1 -> Product2/1
  Gain/1 -> FSphB/1
  Product2/1 -> FSphF/1
  Sum/1 -> Fn/1, Product/2
  dvect/1 -> Gain1/1
  Product/1 -> Product2/2, Gain/1
  Gain1/1 -> Product/1
